simulink model "L150_Path_Follow"  (R2026a)
settings: Solver=VariableStepAuto  StopTime=55.0
undefined symbols (not defined in the file): waypoints
libraries: robotmobilelib x1, simulink x1, robotalgslib x1
settings Model: Creator=hanjiatong  LastModifiedBy=hanjiatong

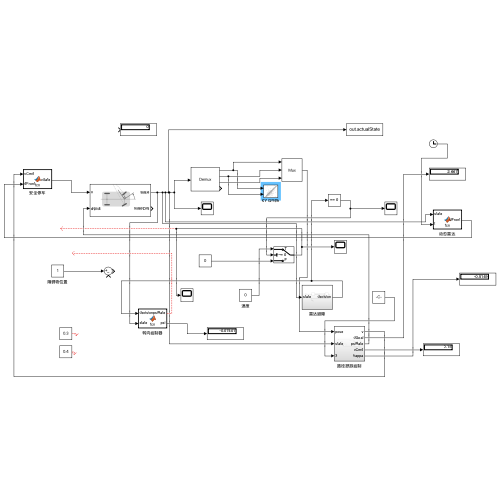
[thumbnail: Simulink's stored preview of the top-level diagram]
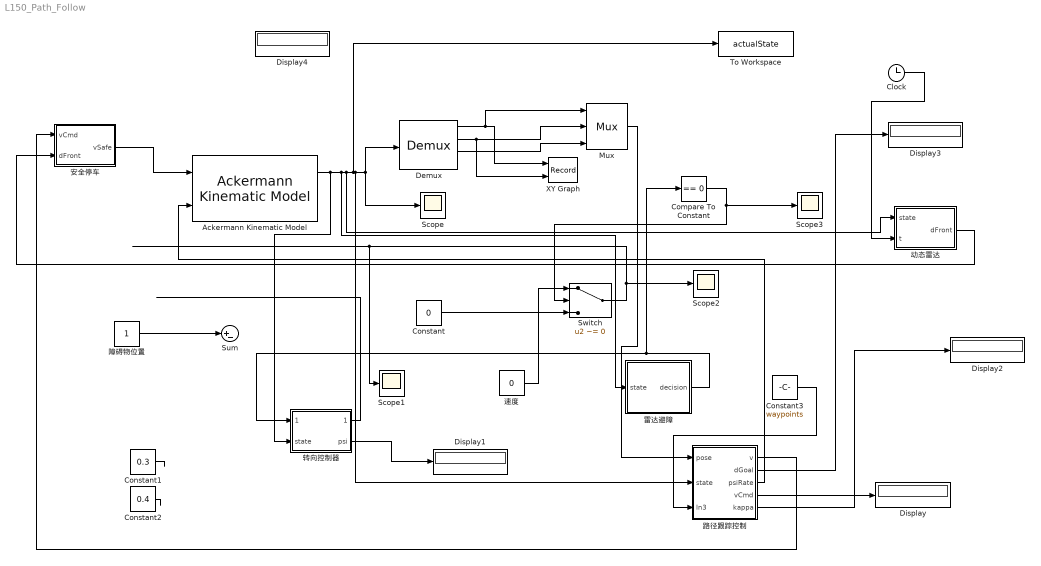
== system L150_Path_Follow ==
  Ackermann Kinematic Model : robotmobilelib/Ackermann Kinematic Model  WheelBase=0.144  VehicleSpeedRange=[-inf inf]  MaxSteeringAngle=pi/4  InitialState=[1; 3; 0; 0]  SimulateUsing=Interpreted execution
  Clock : Clock
  Compare To Constant : simulink/Logic and Bit Operations/Compare To Constant  relop===  const=0  OutDataTypeStr=boolean
  Constant : Constant  Value=0
  Constant1 : Constant  Value=0.3
  Constant2 : Constant  Value=0.4
  Constant3 : Constant  Value=waypoints
  Demux : Demux
      settings: DisplayOption=none
  Display{,1..4} (5 alike) : Display
  Mux : Mux  Inputs=3
  Scope{,1..3} (4 alike) : Scope
      Scope settings: ActiveDisplayYMinimum=-0.19594221664657985  ActiveDisplayYMaximum=1.7514452129987257
      Scope1 settings: ActiveDisplayYMinimum=-1  ActiveDisplayYMaximum=1
      Scope2 settings: ActiveDisplayYMinimum=-0.018749999999999996  ActiveDisplayYMaximum=0.16874999999999998  DataLoggingVariableName=ScopeData2
      Scope3 settings: ActiveDisplayYMinimum=0.33124999999999571  ActiveDisplayYMaximum=1.018749999999998  DataLoggingVariableName=ScopeData3
  Sum : Sum  Inputs=|+-
  Switch : Switch  Criteria=u2 ~= 0  SaturateOnIntegerOverflow=off  InputSameDT=off
  To Workspace : ToWorkspace  VariableName=actualState  SaveFormat=Timeseries  SampleTime=-1
  XY Graph : Record  NumPorts=2.0  FileSettingsInternal="{\"entries\":[{\"content\":{\"excelSettings\":{\"content\":{},\"type\":\"Streamout.ExcelSettings\"},\"parquetSettings\":{\"content\":{},\"type\":\"Streamout.ParquetSettings\"}},\"type\":\"Streamout.FileSettingStorage\",\"uuid\":\"\"}],\"packageUris\":[\"http:\\/\\/schema.mathworks.com\\/mf0\\/streamout_blocks\\/R2020a\"],\"version\":\"1.0\"}"  FrameSettings=[0, 0]  Layout=[1 1]  SignalsInternal="{\"entries\":[{\"content\":{\"signals\":[{\"content\":{\"blockPath\":[],\"dimensions\":[1],\"domain\":\"\",\"lineColor\":\"#a2142f\",\"plots\":[ 1 ],\"port\":1,\"sid\":[\"\"],\"signalID\":1,\"signalName\":\"Demux:1\"},\"type\":\"RecordBlkView.Signal\",\"uuid\":\"\"},{\"content\":{\"blockPath\":[],\"dimensions\":[1],\"domain\":\"\",\"lineColor\":\"#139fff\",\"plots\":[ 1 ],\"port\":2,\"sid\":[\"\"],\"signalID\":2,\"signalName\":\"Demux:2\"},\"type\":\"RecordBlkView.Signal\",\"uuid\":\"\"}]},\"type\":\"RecordBlkView.InputSignals\",\"uuid\":\"\"}],\"packageUris\":[\"http:\\/\\/schema.mathworks.com\\/mf0\\/streamout_blocks\\/R2020a\"],\"version\":\"1.0\"}"  VisualizationBindings="{\"xyplotplugin\":{\"info\":[{\"series\":[{\"bindingParametersList\":[{\"parameter\":\"X-Axis\",\"signalID\":1,\"signalName\":\"Demux:1\"},{\"parameter\":\"Y-Axis\",\"signalID\":2,\"signalName\":\"Demux:2\"}],\"seriesID\":0}],\"subplotID\":1}]}}"  CompatibilityTag=XY
  动态雷达 : MATLAB Function  TreatAsAtomicUnit=on
  安全停车 : MATLAB Function  TreatAsAtomicUnit=on
  路径跟踪控制 : Subsystem
  转向控制器 : MATLAB Function  TreatAsAtomicUnit=on
  速度 : Constant  Value=0
  障碍物位置 : Constant
  雷达避障 : Subsystem
  wires:
  Ackermann Kinematic Model/1 -> 转向控制器/2(state), 动态雷达/1(state), 路径跟踪控制/2(state), Scope/1, Demux/1, To Workspace/1, 雷达避障/1(state)
  Demux/2 -> XY Graph/2, Mux/2
  障碍物位置/1 -> Sum/1
  Switch/1 -> Scope2/1, Scope1/1
  Compare To Constant/1 -> Scope3/1, Switch/2
  速度/1 -> Switch/1
  Constant/1 -> Switch/3
  转向控制器/1(psiRate) -> ?
  转向控制器/2(psi) -> Display1/1
  Constant1/1 -> ?
  Constant2/1 -> ?
  Demux/1 -> Mux/1, XY Graph/1
  Demux/3 -> Mux/3
  雷达避障/1(decision) -> Compare To Constant/1, 转向控制器/1(decision)
  路径跟踪控制/1(v) -> 安全停车/1(vCmd)
  Mux/1 -> 路径跟踪控制/1(pose)
  Constant3/1 -> 路径跟踪控制/3(In3)
  路径跟踪控制/2(dGoal) -> Display3/1
  路径跟踪控制/3(psiRate) -> Ackermann Kinematic Model/2
  路径跟踪控制/4(vCmd) -> Display/1
  路径跟踪控制/5(kappa) -> Display2/1
  Clock/1 -> 动态雷达/2(t)
  动态雷达/1(dFront) -> 安全停车/2(dFront)
  安全停车/1(vSafe) -> Ackermann Kinematic Model/1

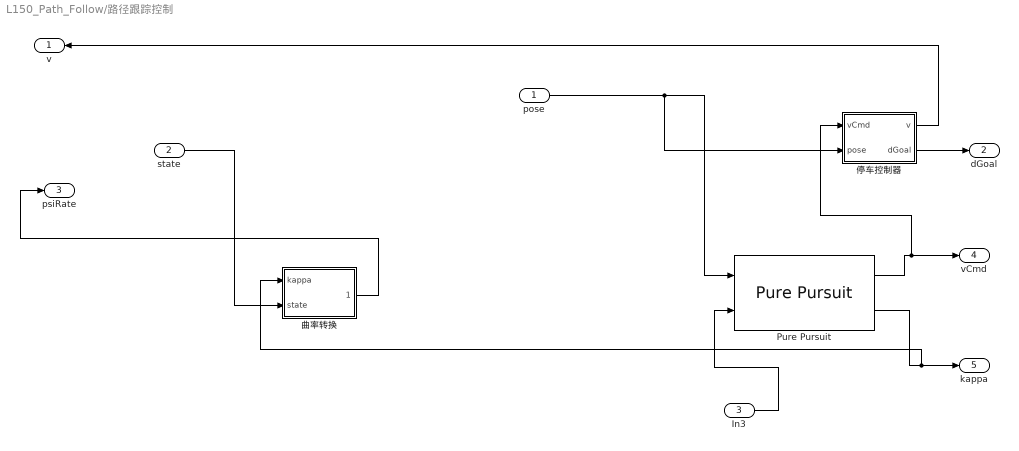
== system L150_Path_Follow/路径跟踪控制 ==
  pose : Inport
  state : Inport  Port=2
  In3 : Inport  Port=3
  Pure Pursuit : robotalgslib/Pure Pursuit  DesiredLinearVelocityPort=off  DesiredLinearVelocity=0.15  MaxCurvature=1/0.96  LookaheadDistancePort=off  LookaheadDistance=0.5  TargetDirPort=off  SimulateUsing=Code generation
      settings: LibrarySourceBlock=navlib/Control Algorithms/Pure Pursuit
  停车控制器 : MATLAB Function  TreatAsAtomicUnit=on
  曲率转换 : MATLAB Function  TreatAsAtomicUnit=on
  v : Outport
  dGoal : Outport  Port=2
  psiRate : Outport  Port=3
  vCmd : Outport  Port=4
  kappa : Outport  Port=5
  wires:
  停车控制器/2(dGoal) -> dGoal/1
  停车控制器/1(v) -> v/1
  曲率转换/1(psiRate) -> psiRate/1
  Pure Pursuit/1 -> vCmd/1, 停车控制器/1(vCmd)
  state/1 -> 曲率转换/2(state)
  In3/1 -> Pure Pursuit/2
  pose/1 -> 停车控制器/2(pose), Pure Pursuit/1
  Pure Pursuit/2 -> kappa/1, 曲率转换/1(kappa)

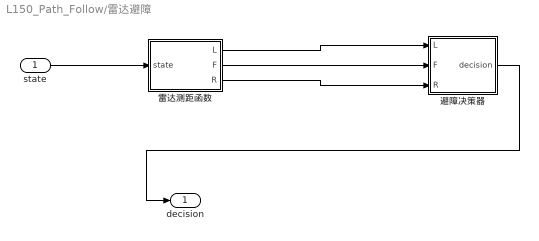
== system L150_Path_Follow/雷达避障 ==
  state : Inport
  " 避障决策器" : MATLAB Function  TreatAsAtomicUnit=on
  雷达测距函数 : MATLAB Function  TreatAsAtomicUnit=on
  decision : Outport
  wires:
  " 避障决策器"/1(decision) -> decision/1
  state/1 -> 雷达测距函数/1(state)
  雷达测距函数/1(L) -> " 避障决策器"/1(L)
  雷达测距函数/3(R) -> " 避障决策器"/3(R)
  雷达测距函数/2(F) -> " 避障决策器"/2(F)

== matlab function L150_Path_Follow/雷达避障/雷达测距函数 ==
  data: state input; L output; F output; R output

function [L, F, R] = fcn(state)
% 输入：小车的状态
% 输出：左、前、右三个方向的障碍物距离

% 在 MATLAB 中执行我们的雷达测距函数
coder.extrinsic('l150ThreeRanges');

% 获取小车的实时位置和朝向
x = state(1);
y = state(2);
theta = state(3);

pose = [x, y, theta];

% 预先声明三个输出都是数值
L = 3.0;
F = 3.0;
R = 3.0;

% 调用刚才写好的三方向雷达函数
[L, F, R] = l150ThreeRanges(pose);

end

== matlab function L150_Path_Follow/转向控制器 ==
  data: decision input; psiRate output; state input; psi output

function [psiRate, psi] = fcn(decision, state)
% 根据避障决定控制前轮转向

% 读取当前前轮转角
psi = state(4);

% 设定目标转角
if decision == 2
    psiTarget = 0.15;    % 左转
elseif decision == 3
    psiTarget = -0.15;   % 右转
else
    psiTarget = 0;       % 回正
end

% 根据转角误差计算转向变化率
error = psiTarget - psi;
psiRate = 2 * error;

% 限制转向速度
psiRate = max(-0.1, min(0.1, psiRate));

end

== matlab function L150_Path_Follow/路径跟踪控制/曲率转换 ==
  data: kappa input; psiRate output; state input

function psiRate = fcn(kappa, state)
% 根据路径曲率计算前轮转向变化率

L = 0.144;              % 轴距
psi = state(4);         % 当前前轮转角

% 根据曲率计算目标转角
psiTarget = atan(L*kappa);

% 限制目标转角
psiTarget = max(-0.15, min(0.15, psiTarget));

% 比例控制
psiRate = 2*(psiTarget-psi);

% 限制转向变化率
psiRate = max(-0.1, min(0.1, psiRate));
end

== matlab function L150_Path_Follow/路径跟踪控制/停车控制器 ==
  data: vCmd input; v output; pose input; dGoal output

function [v, dGoal] = fcn(vCmd, pose)
% 终点停车控制器
% vCmd：Pure Pursuit 给出的速度
% pose：小车当前位置和朝向
% v：最终发送给小车的速度
% dGoal：小车到终点的距离

% 设置终点
goalX = 7;
goalY = 3;

% 获取小车当前位置
x = pose(1);
y = pose(2);

% 计算到终点的距离
dGoal = sqrt((x-goalX)^2 + (y-goalY)^2);

% 判断是否到达终点
if dGoal <= 0.2
    v = 0;
else
    v = vCmd;
end

end

== matlab function L150_Path_Follow/动态雷达 ==
  data: state input; dFront output; t input

function dFront = fcn(state, t)
% 根据当前小车状态和时间进行动态雷达测距

coder.extrinsic('l150DynamicFront');

pose = [state(1), state(2), state(3)];

dFront = 3.0;
dFront = l150DynamicFront(pose, t);

end

== matlab function L150_Path_Follow/安全停车 ==
  data: vCmd input; vSafe output; dFront input

function vSafe = fcn(vCmd, dFront)
% 雷达安全停车控制

if ~isfinite(dFront) || dFront <= 0.7
    vSafe = 0;
else
    vSafe = vCmd;
end

end

== matlab function L150_Path_Follow/雷达避障/ 避障决策器 ==
  data: L input; decision output; F input; R input

function decision = fcn(L, F, R)
% 避障决策器
% 0 = 前方畅通
% 1 = 停车，暂时无法确定安全绕行方向
% 2 = 左侧可以考虑绕行
% 3 = 右侧可以考虑绕行

decision = 1;

% 前方距离足够远
if F > 0.6
    decision = 0;

% 前方存在需要处理的障碍物
elseif L > 0.8 && L > R + 0.1
    decision = 2;

elseif R > 0.8 && R > L + 0.1
    decision = 3;

else
    decision = 1;
end

end
